simulink model "FYP_pwm_model"  (Simulink 7.6)
settings: Solver=FixedStepDiscrete  SolverMode=SingleTasking  StartTime=0.0  StopTime=10.0  FixedStep=0.001  RelTol=1e-3
libraries: dsPICConfigLib x3, dsPICdrivers x2, simulink x1
settings Model: Creator=lab  LastModifiedBy=lab
settings OptimizationCC: OptimizeModelRefInitCode=on
settings HardwareCC: ProdBitPerInt=16  ProdBitPerPointer=16  ProdIntDivRoundTo=Zero  ProdEndianess=LittleEndian  ProdWordSize=16  ProdHWDeviceType=Microchip->dsPIC
settings RTWCC: SystemTargetFile=dsPIC_stf.tlc  TemplateMakefile=dsPIC_gcc.tmf  Description=Embedded Target for Microchip dsPIC33fxx (real-time)  ProcessScript=dsPIC_stf_make_rtw_hook
settings CodeAppCC: IgnoreCustomStorageClasses=off
settings STFCustomTargetCC: ModelReferenceCompliant=off  IncludeMdlTerminateFcn=off  CombineOutputUpdateFcns=on  ERTCustomFileBanners=on  SupportContinuousTime=off  SupportNonInlinedSFcns=off  SystemTargetFile=dsPIC_stf.tlc
settings ERTTargetCC: MultiwordLength=2048  ModelReferenceCompliant=off  ParMdlRefBuildCompliant=off  CompOptLevelCompliant=off  IncludeMdlTerminateFcn=off  ERTFirstTimeCompliant=off  ModelStepFunctionPrototypeControlCompliant=off  CPPClassGenCompliant=off  InlinedParameterPlacement=NonHierarchical  ERTSrcFileBannerTemplate=dsPIC_code_template.cgt  ERTHdrFileBannerTemplate=dsPIC_code_template.cgt  ERTDataSrcFileTemplate=dsPIC_code_template.cgt  ERTDataHdrFileTemplate=dsPIC_code_template.cgt  ERTCustomFileTemplate=dsPIC_main.tlc  ConvertIfToSwitch=off
settings CustomProperty: DataType=string  Value=33FJ64MC802

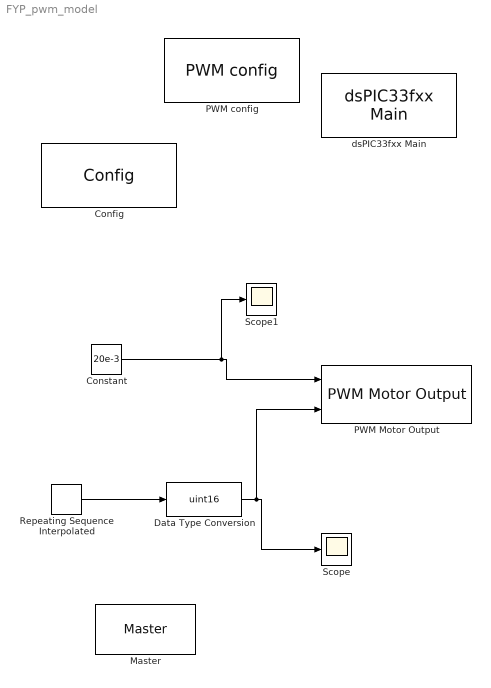
== system FYP_pwm_model ==
  Config : dsPICConfigLib/Config
  Constant : Constant  Value=20e-3  VectorParams1D=off  OutMin=[0]  OutMax=[20e-3]  OutDataTypeStr=uint16  LockScale=on
  Data Type Conversion : DataTypeConversion  OutDataTypeStr=uint16
  Master : dsPICdrivers/Master  Tag=dsPIC_MASTER  Priority=1  TimeStepType=Timer1  picType=33fj64MC802  fcy=6000000  Quartz_33f=12e6  PLLActive_33f=off  fcyDesired_33f=0  tmr1="[1  4999  0]"  tmr1Info="Time Step : 0.001  ;   Error : 0%  PR1=4999"  tmr2345="[0  0  0  0]"  tmr2345cfg=[-1 -1 -1 -1]  IOautoConf=on  typePort="[ 0   0   0   0   0   0   0   0   0   0   0   0   0   0   0   0   0   0   0   0   0   0   0   0   0  11   0   0   0   0   0   0   0   0   0   0   0   0   0   0   0   0   0   0   0   0   0   0   0   0   0   0   0   0   0   0   0   0   0   0   0   0   0   0   0   0   0   0   0   0   0   0   0   0   0   0   0   0   0   0   0   0   0   0   0   0   0   0   0   0   0   0   0   0   0   0   0   0   0   0   0   0   0   0   0   0   0   0   0   0   0   0 ]"  TRIS="[ 65535  65535  65535  65535  65535  65535  65535 ]"  ADPCFG=0  MasterBusyPort=None  MasterOverloadPort=None  FOSC=Quartz (XT - HS)  ClockSwitchMonitor=Both disabled  TempProtection_33f=TEMP_ON  FPBOR=<empty>  PWRT=disable  MCLR=<empty>  ICD=ICS_PGD1  JTAGEN=JTAGEN_OFF  PowerSave=off  OverrideFcy=on  NewFcy=5e6  PR2345="[65535  65535  65535  65535]"
  PWM Motor Output : dsPICdrivers/Peripheral I//O/PWM Motor Output  Tag=dsPIC_PWM_Motor  Priority=5  PWMref=2  PWM12=2  InputEnableChk=off  InputPeriodeChk=on  Channel=[1 ]  TPeriode=20E-3  PrescalerValue=4  PeriodeInteger=12500  MaxName='PWM2'  Centered=on  HChannelON=off  Info="Nbr Bits : 14.6096  ||  PWM2 = 25000  ||  Prescaler = 4"  Delay=0  IntPriority=5  nbrPwmChannelPIC=1  Status=OK  DeadTimePrescaleA=1e-6  DeadTimePrescaleB=0  DeadTimeInfo="Dead Time A = 1e-006  ||  Dead Time B = 0"  DTPWM1a=Prescaler A  DTPWM1i=Prescaler A  DTPWM2a=Prescaler A  DTPWM2i=Prescaler A  DTPWM3a=Prescaler A  DTPWM3i=Prescaler A  DTPWM4a=Prescaler A  DTPWM4i=Prescaler A  DTCON1=5  DTCON2=0
  PWM config : dsPICConfigLib/PWM config  Priority=-19  PWMSEL=2  PTPER=159999  PDC1=3204780  PDC4=1600  PMOD1=complementary output mode  PMOD2=complementary output mode  PMOD3=complementary output mode  PMOD4=complementary output mode  PEN4H=off  PEN3H=off  PEN2H=off  PEN1H=on  PEN4L=off  PEN3L=off  PEN2L=off  PEN1L=on  IUE=off  OSYNC=Output overrides via the PxOVDCON(1) register occur on the next TCY boundary  UDIS=off  PWMINTEN=off  PWMINTP=0  SEVTDIR=Trigger when PWM time base is counting up  SEVTCMP=100000  PTEN=off  PTSIDL=off  PTOPS=1  PTCKPS=input clock period is TCY (1:1 prescale)  PTMOD=Free Running mode  PTFREQ=25  PDC1P=2003  PDC2P="Apply Positive dead time  for all output modes"  PDC3P=off  PDC4P=1  PWMPIN=Control pin state at reset by the module  HPOL=Ative Low  LPOL=Ative Low  DTBPS=Clock period for Dead Time Unit B is TCY  DTB=397  DTAPS=Clock period for Dead Time Unit A is TCY  DTA=0  DTS4A=Dead time provided from Unit A  DTS4I=Dead time provided from Unit A  DTS3A=Dead time provided from Unit A  DTS3I=Dead time provided from Unit A  DTS2A=Dead time provided from Unit A  DTS2I=Dead time provided from Unit A  DTS1A=Dead time provided from Unit A  DTS1I=Dead time provided from Unit A  FAOV4H=Drive PWM output pin Inactive on an external fault input event  FAOV3H=Drive PWM output pin Inactive on an external fault input event  FAOV2H=Drive PWM output pin Inactive on an external fault input event  FAOV1H=Drive PWM output pin Inactive on an external fault input event  FAOV4L=Drive PWM output pin Inactive on an external fault input event  FAOV3L=Drive PWM output pin Inactive on an external fault input event  FAOV2L=Drive PWM output pin Inactive on an external fault input event  FAOV1L=Drive PWM output pin Inactive on an external fault input event  FLTAM=Fault A input pin latches all control pins to the programmed states in PxFLTACON<15:8>  FAEN4=off  FAEN3=off  FAEN2=off  FAEN1=off  FBOV4H=Drive PWM output pin Inactive on an external fault input event  FBOV3H=Drive PWM output pin Inactive on an external fault input event  FBOV2H=Drive PWM output pin Inactive on an external fault input event  FBOV1H=Drive PWM output pin Inactive on an external fault input event  FBOV4L=Drive PWM output pin Inactive on an external fault input event  FBOV3L=Drive PWM output pin Inactive on an external fault input event  FBOV2L=Drive PWM output pin Inactive on an external fault input event  FBOV1L=Drive PWM output pin Inactive on an external fault input event  FLTBM=Fault B input pin latches all control pins to the programmed states in PxFLTACON<15:8>  FBEN4=off  FBEN3=off  FBEN2=off  FBEN1=off  POVD4H=off  POUT4H=Drive PWM4H Inactive when POVD4H bit is cleared  POVD4L=off  POUT4L=Drive PWM4L Inactive when POVD4L bit is cleared  POVD3H=off  POUT3H=Drive PWM3H Inactive when POVD3H bit is cleared  POVD3L=off  POUT3L=Drive PWM3L Inactive when POVD3L bit is cleared  POVD2H=off  POUT2H=Drive PWM2H Inactive when POVD2H bit is cleared  POVD2L=off  POUT2L=Drive PWM2L Inactive when POVD2L bit is cleared  POVD1H=off  POUT1H=Drive PWM1H Inactive when POVD1H bit is cleared  POVD1L=off  POUT1L=Drive PWM1L Inactive when POVD1L bit is cleared
  Repeating Sequence Interpolated : simulink/Sources/Repeating Sequence Interpolated  SystemSampleTime=-1  OutValues=[1 0 1 0 1].'  TimeValues=[0 0.8 1 1.2 2].'  LookUpMeth=Interpolation-Use End Values  tsamp=0.01  OutMin=[]  OutMax=[]  OutDataTypeStr=uint16  OutputDataTypeScalingMode=uint16  OutDataType=fixdt(0,8)  OutScaling=2^-10
  Scope : Scope
      settings: TickLabels=on  TimeRange=5  Decimation=2  SampleInput=on  SampleTime=0.01
  Scope1 : Scope
      settings: TickLabels=on  TimeRange=5  YMin=-1  YMax=0.04  Decimation=2  SampleInput=on  SampleTime=0.01
  dsPIC33fxx Main : dsPICConfigLib/dsPIC33fxx Main  Priority=-50  PICTYPE=33FJ64MC802  timer=Timer1  OscSrcSel=Primary oscillator (XT HS EC)  Fin=8e6  Fcy=4000000  ReqLpTm=1  PR1=4000  IESO=Enabled  Temperature=Disabled  ClockSwi=Both enabled  Osc2=Digital I/O  OscSel=External clock  FICD=Use PGC1/EMUC1 and PGD1/EMUD1  Wdt=Disabled  WinWdt=Disabled  WdtPre=1:32  WdtPost=1:1  HSCP=code protect off  CodeProtect=Disabled  WriteProtect=Disabled  PLLDIV=0  PLLPRE=0  PLLPOST=0  TMR1PRESCL=0
  wires:
  Repeating Sequence Interpolated/1 -> Data Type Conversion/1
  Data Type Conversion/1 -> Scope/1, PWM Motor Output/2
  Constant/1 -> PWM Motor Output/1, Scope1/1
